simulink model "sf_states_when_enabling"  (R2025b)
settings: Solver=FixedStepDiscrete  StartTime=0.0  StopTime=50.0  FixedStep=1  RelTol=1e-3  EnableMultiTasking=on
settings Model: Creator=The MathWorks, Inc.  LastModifiedBy=The MathWorks, Inc.
settings SolverCC: AlgebraicLoopSolver=TrustRegion
settings DataIOCC: LimitDataPoints=on  SaveFormat=Array  ReturnWorkspaceOutputs=off
settings OptimizationCC: ReuseModelBlockBuffer=off  ExpressionDepthLimit=2147483647.0  LifeSpan=inf
settings DebuggingCC: UnderspecifiedInitializationDetection=Classic  MergeDetectMultiDrivingBlocksExec=none  SolverPrmCheckMsg=warning  FcnCallInpInsideContextMsg=warning  UnconnectedInputMsg=warning  UnconnectedOutputMsg=warning  UnconnectedLineMsg=warning  StateNameClashWarn=warning  SFUnexpectedBacktrackingDiag=warning  SFNoUnconditionalDefaultTransitionDiag=warning  SFExecutionAtInitializationDiag=none  ArithmeticOperatorsInVariantConditions=warning
settings HardwareCC: ProdBitPerPointer=32.0  ProdBitPerSizeT=32.0  ProdBitPerPtrDiffT=32.0  ProdLargestAtomicFloat=None  ProdIntDivRoundTo=Undefined  ProdEndianess=Unspecified  ProdWordSize=32.0  ProdHWDeviceType=32-bit Generic
settings ModelReferenceCC: EnableRefExpFcnMdlSchedulingChecks=on  PropagateSignalLabelsOutOfModel=off
settings SFSimCC: SimUseLocalCustomCode=off  SimParseCustomCode=off
settings RTWCC: RTWUseLocalCustomCode=off  GPUComputeCapability=3.5
settings CodeAppCC: StateflowObjectComments=on
settings GRTTargetCC: TargetLangStandard=C89/C90 (ANSI)  CombineOutputUpdateFcns=off  GRTInterface=on
settings ConfigComp: CovMetricSettings=dw  CovSaveCumulativeToWorkspaceVar=on  CovSaveSingleToWorkspaceVar=on  CovExternalEMLEnable=off

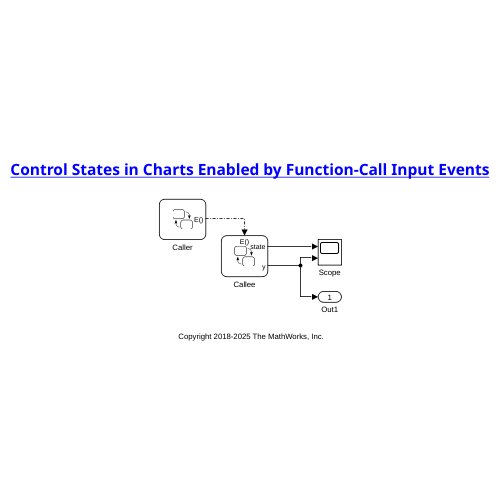
[thumbnail: Simulink's stored preview of the top-level diagram]
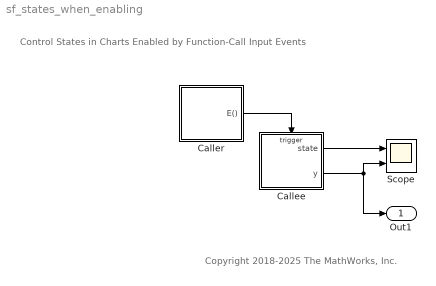
== system sf_states_when_enabling ==
  note: Copyright 2018-2025 The MathWorks, Inc.
  note: Control States in Charts Enabled by Function-Call Input Events
  Callee : Stateflow chart  TreatAsAtomicUnit=on
  Caller : Stateflow chart  TreatAsAtomicUnit=on
  Scope : Scope  NumInputPorts=2
      settings: ActiveDisplayYMinimum=0.875  ActiveDisplayYMaximum=2.125
  Out1 : Outport  VectorParamsAs1DForOutWhenUnconnected=off
  wires:
  Caller/1(E()) -> Callee/Trigger
  Callee/2(y) -> Scope/2, Out1/1
  Callee/1(state) -> Scope/1

== stateflow chart sf_states_when_enabling/Caller ==
  state A
    bind: E;
    en,du: send(E);
  state B
  (default) -> A
  A -> B : after(10,tick)
  B -> A : after(10,tick)
  events: E output FUNCTION_CALL_EVENT

== stateflow chart sf_states_when_enabling/Callee ==
  state C
    y++;
  state D
    y++;
  (default) -> C
  C -> D : [y>0]
  data: state output Enum: CalleeModeType; y output double
  events: E input FUNCTION_CALL_EVENT
